simulink model "scheme_L2"  (R2025b)
settings: Solver=VariableStepAuto  StartTime=0.0  StopTime=10.0  MaxStep=0.005  RelTol=1e-3
settings Model: Creator=student  LastModifiedBy=arina

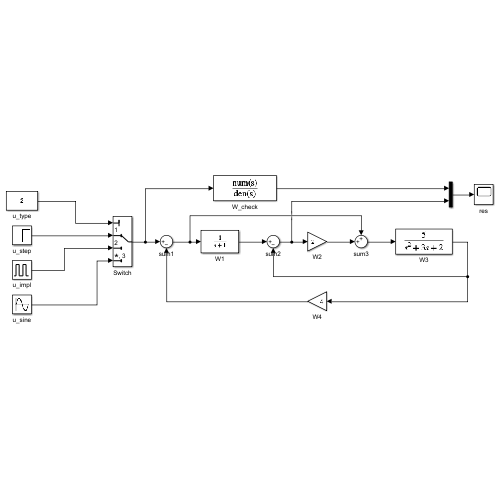
[thumbnail: Simulink's stored preview of the top-level diagram]
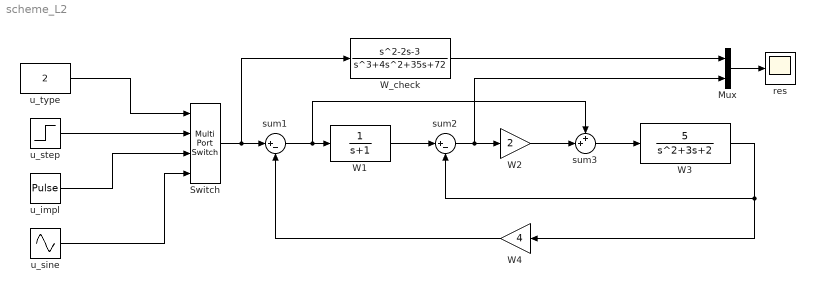
== system scheme_L2 ==
  Mux : Mux  Inputs=2
  Switch : MultiPortSwitch
  W1 : TransferFcn  Denominator=[1 1]
  W2 : Gain  Gain=2
  W3 : TransferFcn  Numerator=[5]  Denominator=[1 3 2]
  W4 : Gain  Gain=4
  W_check : TransferFcn  Numerator=[1 -2 -3]  Denominator=[1 4 35 72]
  res : Scope
      settings: ActiveDisplayYMinimum=-0.2269610552536156  ActiveDisplayYMaximum=0.23143006826526677
  sum1 : Sum  Inputs=|+-
  sum2 : Sum  Inputs=|+-
  sum3 : Sum  Inputs=++|
  u_impl : DiscretePulseGenerator  PulseType=Time based  Amplitude=20  Period=20  PulseWidth=0.2  PhaseDelay=2
  u_sine : Sin  Frequency=3  SampleTime=0
  u_step : Step  SampleTime=0
  u_type : Constant  Value=2
  wires:
  u_type/1 -> Switch/1
  u_step/1 -> Switch/2
  u_impl/1 -> Switch/3
  u_sine/1 -> Switch/4
  Switch/1 -> sum1/1, W_check/1
  sum1/1 -> W1/1, sum3/1
  W1/1 -> sum2/1
  sum2/1 -> W2/1, Mux/2
  W2/1 -> sum3/2
  sum3/1 -> W3/1
  W3/1 -> W4/1, sum2/2
  W4/1 -> sum1/2
  W_check/1 -> Mux/1
  Mux/1 -> res/1
